simulink library "Lib_Piccolo"  (R2018b)
settings: Solver=VariableStepAuto  StartTime=0.0  StopTime=10.0  RelTol=1e-3
values from neighbouring files (symbols this model uses):
  AccelErrInt2Brakes = 0.15    [SimulationControlConfig16P.m]    (also in SimulationControlConfig16P_LEGACY.m; SimulationControlConfigTAILLESS.m = 0.2; SimulationControlConfigUTAIL.m = 0.2)
  AileronMax = 25    [SimulationControlConfig16P.m]    (also in SimulationControlConfig16P_LEGACY.m; SimulationControlConfigTAILLESS.m; SimulationControlConfigUTAIL.m)
  AileronPower = 0.00268    [SimulationControlConfig16P.m]    (also in SimulationControlConfig16P_LEGACY.m; SimulationControlConfigTAILLESS.m; SimulationControlConfigUTAIL.m)
  AileronSurfaceMax = 45    [SimulationControlConfig16P.m]    (also in SimulationControlConfig16P_LEGACY.m)
  AileronTrim = 0    [SimulationControlConfig16P.m]    (also in SimulationControlConfig16P_LEGACY.m; SimulationControlConfigTAILLESS.m; SimulationControlConfigUTAIL.m)
  Alt = 1000 + TerrainHeight    [SimulationStateConfig.m]
  AltCruise_m = testPlans(testIndx).terrainElevation * 0.3048 + 200    [SimulationControlConfig16P.m]    (also in SimulationControlConfigTAILLESS.m = 1083; SimulationControlConfigUTAIL.m = testPlans(testIndx).terrainElevation * 0.3048 + 152)
  AltitudeRate2PitchCmdIntegratorInit = 0.1    [SimulationControlPre.m]
  AltMax = 10000    [SimulationControlConfig16P.m]    (also in SimulationControlConfig16P_LEGACY.m; SimulationControlConfigTAILLESS.m; SimulationControlConfigUTAIL.m)
  AltMaxAccel = 1.25    [SimulationControlConfig16P.m]    (also in SimulationControlConfig16P_LEGACY.m = 0.9; SimulationControlConfigTAILLESS.m = 1.7; SimulationControlConfigUTAIL.m = 2)
  AltMin = 0    [SimulationControlConfig16P.m]    (also in SimulationControlConfig16P_LEGACY.m; SimulationControlConfigTAILLESS.m; SimulationControlConfigUTAIL.m)
  AltRateCmd2Pitch = 0.50    (= 0.5)    [SimulationControlConfig16P.m]    (also in SimulationControlConfig16P_LEGACY.m = 0.6; SimulationControlConfigTAILLESS.m = 0.2; SimulationControlConfigUTAIL.m = 0.3)
  AltRateError2Pitch = 0.40    (= 0.4)    [SimulationControlConfig16P.m]    (also in SimulationControlConfig16P_LEGACY.m; SimulationControlConfigTAILLESS.m = 0.55; SimulationControlConfigUTAIL.m = 0.55)
  AltRateErrorInt2Pitch = 0.50    (= 0.5)    [SimulationControlConfig16P.m]    (also in SimulationControlConfig16P_LEGACY.m = 0.45; SimulationControlConfigTAILLESS.m; SimulationControlConfigUTAIL.m = 0.75)
  AltRateLpfCutOff = 3    [SimulationControlConfig16P.m]    (also in SimulationControlConfig16P_LEGACY.m; SimulationControlConfigTAILLESS.m = 2; SimulationControlConfigUTAIL.m = 2)
  AutoNosegear2Rudder = 26    [SimulationControlConfig16P.m]    (also in SimulationControlConfig16P_LEGACY.m; SimulationControlConfigTAILLESS.m = 25.2; SimulationControlConfigUTAIL.m = 14)
  b = 5.54    [SimulationControlConfig16P.m]    (also in SimulationControlConfig16P_LEGACY.m; SimulationControlConfigTAILLESS.m = 2.37; SimulationControlConfigUTAIL.m = 2.37)
  Bank2AileronIntegratorInit = 0    [SimulationControlPre.m]
  BankMax_User = BankMax_User/180*pi    (= 0.523598775598)    [SimulationControlConfig16P.m]    (also in SimulationControlConfig16P_LEGACY.m; SimulationControlConfigTAILLESS.m = 0.610865238198; SimulationControlConfigUTAIL.m = 0.628318530718)
  baseLegFlaps = 20    [SimulationControlConfig16P.m]    (also in SimulationControlConfig16P_LEGACY.m = 0; SimulationControlConfigTAILLESS.m = 15; SimulationControlConfigUTAIL.m = 10)
  C = GeneticOpt.C    [SimulationCostFunction.m]
  c = Sw/b    (= 0.841696750903)    [SimulationControlConfig16P.m]    (also in SimulationControlConfig16P_LEGACY.m; SimulationControlConfigTAILLESS.m = 0.354008438819; SimulationControlConfigUTAIL.m = 0.354008438819)
  cell2WheelFactorMG = 5.98    [SimulationSensorConfig16P_LEGACY.m]
  cell2WheelFactorNG = 1    [SimulationSensorConfig16P_LEGACY.m]
  cellSatMaxMG = 15000    [SimulationSensorConfig16P.m]    (also in SimulationSensorConfig16P_LEGACY.m; SimulationSensorConfigTAILLESS7P.m; SimulationSensorConfigUTAIL7P.m)
  cellSatMaxNG = 1000    [SimulationSensorConfig16P.m]    (also in SimulationSensorConfig16P_LEGACY.m; SimulationSensorConfigTAILLESS7P.m; SimulationSensorConfigUTAIL7P.m)
  cellSatMinMG = -15000    [SimulationSensorConfig16P.m]    (also in SimulationSensorConfig16P_LEGACY.m; SimulationSensorConfigTAILLESS7P.m; SimulationSensorConfigUTAIL7P.m)
  cellSatMinNG = -1000    [SimulationSensorConfig16P.m]    (also in SimulationSensorConfig16P_LEGACY.m; SimulationSensorConfigTAILLESS7P.m; SimulationSensorConfigUTAIL7P.m)
  CL_Limit = CL_Max    (= 0.54)    [SimulationControlConfig16P.m]    (also in SimulationControlConfig16P_LEGACY.m; SimulationControlConfigTAILLESS.m; SimulationControlConfigUTAIL.m = 0.53)
  CL_Max = 0.54    [SimulationControlConfig16P.m]    (also in SimulationControlConfig16P_LEGACY.m; SimulationControlConfigTAILLESS.m; SimulationControlConfigUTAIL.m = 0.53)
  CL_Max_Nom = 0.465    [SimulationControlConfig16P.m]    (also in SimulationControlConfig16P_LEGACY.m; SimulationControlConfigTAILLESS.m = 0.39; SimulationControlConfigUTAIL.m)
  CL_Min = 0    [SimulationControlConfig16P.m]    (also in SimulationControlConfig16P_LEGACY.m; SimulationControlConfigTAILLESS.m; SimulationControlConfigUTAIL.m)
  ClimbMaxFraction = 0.35    [SimulationControlConfig16P.m]    (also in SimulationControlConfig16P_LEGACY.m = 0.24; SimulationControlConfigTAILLESS.m = 0.19; SimulationControlConfigUTAIL.m = 0.21)
  ClimboutMaxBank = 7.0    (= 7)    [SimulationControlConfig16P.m]    (also in SimulationControlConfig16P_LEGACY.m; SimulationControlConfigTAILLESS.m = 5; SimulationControlConfigUTAIL.m)
  ClimboutTimer = 7.0    (= 7)    [SimulationControlConfig16P.m]    (also in SimulationControlConfig16P_LEGACY.m; SimulationControlConfigTAILLESS.m; SimulationControlConfigUTAIL.m)
  dCl_per_dFlap = 0.005581818    [SimulationControlConfig16P.m]    (also in SimulationControlConfig16P_LEGACY.m = 0; SimulationControlConfigTAILLESS.m = 0; SimulationControlConfigUTAIL.m = 0)
  DecelerationCmd = 3.1    [SimulationControlConfig16P.m]    (also in SimulationControlConfig16P_LEGACY.m; SimulationControlConfigTAILLESS.m = 0.1; SimulationControlConfigUTAIL.m = 0.1)
  DeRotateLogicEndTimer = abs((NoseDownLimit_Deg-1)/DeRotateRamp_Dps)    [SimulationControlConfig16P.m]    (also in SimulationControlConfig16P_LEGACY.m; SimulationControlConfigTAILLESS.m; SimulationControlConfigUTAIL.m)
  DeRotateLogicHoldNoseUpTimer = 0.1    [SimulationControlConfig16P.m]    (also in SimulationControlConfig16P_LEGACY.m; SimulationControlConfigTAILLESS.m; SimulationControlConfigUTAIL.m)
  DeRotateLogicTimerTimeout = 2    [SimulationControlConfig16P.m]    (also in SimulationControlConfig16P_LEGACY.m; SimulationControlConfigTAILLESS.m; SimulationControlConfigUTAIL.m)
  DeRotateLowerCmdSaturation = 0    [SimulationControlConfig16P.m]    (also in SimulationControlConfig16P_LEGACY.m; SimulationControlConfigTAILLESS.m; SimulationControlConfigUTAIL.m)
  DeRotateRamp_Dps = 3    [SimulationControlConfig16P.m]    (also in SimulationControlConfig16P_LEGACY.m; SimulationControlConfigTAILLESS.m = 8; SimulationControlConfigUTAIL.m = 8)
  DeRotateUpperCmdSaturation = 7    [SimulationControlConfig16P.m]    (also in SimulationControlConfig16P_LEGACY.m; SimulationControlConfigTAILLESS.m; SimulationControlConfigUTAIL.m)
  DescentMaxFraction = 0.22    [SimulationControlConfig16P.m]    (also in SimulationControlConfig16P_LEGACY.m = 0.2; SimulationControlConfigTAILLESS.m = 0.17; SimulationControlConfigUTAIL.m = 0.17)
  DesktopSimTerrainOffset_m = 0.406    [SimulationAircraftConfig.m]
  downwindFlaps = 0    [SimulationControlConfig16P.m]    (also in SimulationControlConfig16P_LEGACY.m; SimulationControlConfigTAILLESS.m; SimulationControlConfigUTAIL.m)
  DP_init = 0.5*1.225*V_init^2    [SimulationControlConfig16P.m]    (also in SimulationControlConfig16P_LEGACY.m; SimulationControlConfigTAILLESS.m; SimulationControlConfigUTAIL.m)
  dscNoiseMG = 1    [SimulationSensorConfig16P_LEGACY.m]
  dscNoiseNG = 0.25    [SimulationSensorConfig16P_LEGACY.m]
  DSCnumBits = 24    [SimulationSensorConfig16P.m]    (also in SimulationSensorConfig16P_LEGACY.m; SimulationSensorConfigTAILLESS7P.m; SimulationSensorConfigUTAIL7P.m)
  DSCRangeMaxMG = 15000    [SimulationSensorConfig16P.m]    (also in SimulationSensorConfig16P_LEGACY.m; SimulationSensorConfigTAILLESS7P.m; SimulationSensorConfigUTAIL7P.m)
  DSCRangeMaxNG = 1000    [SimulationSensorConfig16P.m]    (also in SimulationSensorConfig16P_LEGACY.m; SimulationSensorConfigTAILLESS7P.m; SimulationSensorConfigUTAIL7P.m)
  DSCRangeMinMG = -15000    [SimulationSensorConfig16P.m]    (also in SimulationSensorConfig16P_LEGACY.m; SimulationSensorConfigTAILLESS7P.m; SimulationSensorConfigUTAIL7P.m)
  DSCRangeMinNG = -1000    [SimulationSensorConfig16P.m]    (also in SimulationSensorConfig16P_LEGACY.m; SimulationSensorConfigTAILLESS7P.m; SimulationSensorConfigUTAIL7P.m)
  dt = DLLSim.dt    [SimulationTimeStep.m]    (also in SimulationTrim.m = 0.02)
  EarlyTouchdownThreshold = 3.0    (= 3)    [SimulationControlConfig16P.m]    (also in SimulationControlConfig16P_LEGACY.m; SimulationControlConfigTAILLESS.m = 2.2; SimulationControlConfigUTAIL.m = 2.5)
  ElevatorDeflectionRate = 15    [SimulationControlConfig16P.m]    (also in SimulationControlConfig16P_LEGACY.m = 12; SimulationControlConfigTAILLESS.m = 10; SimulationControlConfigUTAIL.m = 12)
  ElevatorMax = 25    [SimulationControlConfig16P.m]    (also in SimulationControlConfig16P_LEGACY.m; SimulationControlConfigTAILLESS.m; SimulationControlConfigUTAIL.m)
  ElevatorPower = -0.002209    [SimulationControlConfig16P.m]    (also in SimulationControlConfig16P_LEGACY.m; SimulationControlConfigTAILLESS.m = -0.002956; SimulationControlConfigUTAIL.m = -0.00205983)
  ElevatorTrim = -3.5    [SimulationControlConfig16P.m]    (also in SimulationControlConfig16P_LEGACY.m; SimulationControlConfigTAILLESS.m = -6; SimulationControlConfigUTAIL.m = -8)
  elevonBias = 0    [SimulationControlConfig16P.m]    (also in SimulationControlConfig16P_LEGACY.m; SimulationControlConfigTAILLESS.m; SimulationControlConfigUTAIL.m)
  Enable_TAS_Protection = 0    [SimulationControlConfig16P.m]    (also in SimulationControlConfig16P_LEGACY.m; SimulationControlConfigTAILLESS.m; SimulationControlConfigUTAIL.m)
  EnableCrossTrackAbort = 1    [SimulationControlConfig16P.m]    (also in SimulationControlConfigTAILLESS.m; SimulationControlConfigUTAIL.m)
  EnergyBandwidth = 0.02    [SimulationControlConfig16P.m]    (also in SimulationControlConfig16P_LEGACY.m; SimulationControlConfigTAILLESS.m = 0.06; SimulationControlConfigUTAIL.m = 0.06)
  EngineLhFuelCut = 0    [SimulationAircraftConfig.m]
  EngineRhFuelCut = 0    [SimulationAircraftConfig.m]
  FastThrottleRate = 0.075    [SimulationControlConfig16P.m]    (also in SimulationControlConfig16P_LEGACY.m = 0.05; SimulationControlConfigTAILLESS.m = 0.1; SimulationControlConfigUTAIL.m = 0.1)
  FilterWarmUpTime = 2    [SimulationSensorConfig16P.m]    (also in SimulationSensorConfig16P_LEGACY.m; SimulationSensorConfigTAILLESS7P.m; SimulationSensorConfigUTAIL7P.m)
  finalApproachFlaps = 20    [SimulationControlConfig16P.m]    (also in SimulationControlConfig16P_LEGACY.m = 0; SimulationControlConfigTAILLESS.m = 22; SimulationControlConfigUTAIL.m = 10)
  FinalDescentSlope_Deg = testPlans(testIndx).descentSlope    [SimulationControlConfig16P.m]    (also in SimulationControlConfig16P_LEGACY.m; SimulationControlConfigTAILLESS.m; SimulationControlConfigUTAIL.m)
  flapMax = 0    [SimulationControlConfig16P.m]    (also in SimulationControlConfig16P_LEGACY.m; SimulationControlConfigTAILLESS.m; SimulationControlConfigUTAIL.m)
  flapRate = 7.5    [SimulationControlConfig16P.m]    (also in SimulationControlConfig16P_LEGACY.m; SimulationControlConfigTAILLESS.m = 6.6; SimulationControlConfigUTAIL.m)
  FlareHeight = 5    [SimulationControlConfig16P.m]    (also in SimulationControlConfig16P_LEGACY.m = 4.8; SimulationControlConfigTAILLESS.m = 2.5; SimulationControlConfigUTAIL.m = 2)
  FlareVerticalRate_mps = -0.4    [SimulationControlConfig16P.m]    (also in SimulationControlConfig16P_LEGACY.m = -0.5; SimulationControlConfigTAILLESS.m = -0.15; SimulationControlConfigUTAIL.m = -0.15)
  Fp_Aileron = 0.55*2*pi*RollRateLpfCutoff*dt    [SimulationControlConfig16P.m]    (also in SimulationControlConfig16P_LEGACY.m; SimulationControlConfigTAILLESS.m; SimulationControlConfigUTAIL.m)
  Fp_Alt = 0.55*AltBandwidth    (= 0.099)    [SimulationControlConfig16P.m]    (also in SimulationControlConfig16P_LEGACY.m; SimulationControlConfigTAILLESS.m = 0.587477826221; SimulationControlConfigUTAIL.m = 0.69115038379)
  Fp_AltRate = 0.55*2*pi*AltRateLpfCutOff*dt    [SimulationControlConfig16P.m]    (also in SimulationControlConfig16P_LEGACY.m; SimulationControlConfigTAILLESS.m; SimulationControlConfigUTAIL.m)
  Fp_Elevator = 0.55*2*pi*PitchRateLpfCutoff*dt    [SimulationControlConfig16P.m]    (also in SimulationControlConfig16P_LEGACY.m; SimulationControlConfigTAILLESS.m; SimulationControlConfigUTAIL.m)
  Fp_Energy = 0.55*2*pi*EnergyBandwidth    (= 0.069115038379)    [SimulationControlConfig16P.m]    (also in SimulationControlConfig16P_LEGACY.m; SimulationControlConfigTAILLESS.m = 0.207345115137; SimulationControlConfigUTAIL.m = 0.207345115137)
  Fp_Energy2 = 0.55*2*pi*EnergyBandwidth*dt    [SimulationControlConfig16P.m]    (also in SimulationControlConfig16P_LEGACY.m; SimulationControlConfigTAILLESS.m; SimulationControlConfigUTAIL.m)
  Fp_Pitch = 0.55*2*pi*PitchBandwidth    (= 2.76460153516)    [SimulationControlConfig16P.m]    (also in SimulationControlConfig16P_LEGACY.m = 3.11017672705; SimulationControlConfigTAILLESS.m = 3.80132711084; SimulationControlConfigUTAIL.m = 2.41902634326)
  Fp_Pitch_2 = 0.55*2*pi*PitchBandwidth*dt    [SimulationControlConfig16P.m]    (also in SimulationControlConfig16P_LEGACY.m; SimulationControlConfigTAILLESS.m; SimulationControlConfigUTAIL.m)
  Fp_Roll = RollBandwidth^2    (= 1)    [SimulationControlConfig16P.m]    (also in SimulationControlConfig16P_LEGACY.m = 1.44; SimulationControlConfigTAILLESS.m; SimulationControlConfigUTAIL.m)
  Fp_Rudder = 0.55*2*pi*YawRateLpfCutoff*dt    [SimulationControlConfig16P.m]    (also in SimulationControlConfig16P_LEGACY.m; SimulationControlConfigTAILLESS.m; SimulationControlConfigUTAIL.m)
  Fp_TAS = 0.55*2*pi*TASBandwidth    (= 0.103672557568)    [SimulationControlConfig16P.m]    (also in SimulationControlConfig16P_LEGACY.m; SimulationControlConfigTAILLESS.m = 0.172787595947; SimulationControlConfigUTAIL.m = 0.172787595947)
  Fp_TAS_Filter = 2*pi*TasLpfCutoff*dt    [SimulationControlConfig16P.m]    (also in SimulationControlConfig16P_LEGACY.m; SimulationControlConfigTAILLESS.m; SimulationControlConfigUTAIL.m)
  Fp_Turn = 0.55*2*pi*TurnErrLPFcutoff    (= 0.0345575191895)    [SimulationControlConfig16P.m]    (also in SimulationControlConfig16P_LEGACY.m; SimulationControlConfigTAILLESS.m = 0.172787595947; SimulationControlConfigUTAIL.m = 0.172787595947)
  Fp_TurnDerr = 0.55*2*pi*TurnDerivativeLPFcutoff    (= 0.0345575191895)    [SimulationControlConfig16P.m]    (also in SimulationControlConfig16P_LEGACY.m; SimulationControlConfigTAILLESS.m = 0.172787595947; SimulationControlConfigUTAIL.m = 0.172787595947)
  FTV = 3    [SimulationAircraftConfig.m]
  ftvStaticPositionError = 1/1.18    (= 0.847457627119)    [SimulationSensorConfig16P.m]    (also in SimulationSensorConfig16P_LEGACY.m; SimulationSensorConfigTAILLESS7P.m = 1; SimulationSensorConfigUTAIL7P.m = 1)
  g = 9.81    [SimulationStateConfig.m]
  GustSpd_Kts = testPlans(testIndx).gustSpd    [SimulationStateConfig.m]
  GustTriggerVal = testPlans(testIndx).gustTriggerVal    [SimulationStateConfig.m]
  HeadingErr2TurnRate = 0.5    [SimulationControlConfig16P.m]    (also in SimulationControlConfig16P_LEGACY.m; SimulationControlConfigTAILLESS.m; SimulationControlConfigUTAIL.m)
  HeadingErrDer2TurnRate = 0.3    [SimulationControlConfig16P.m]    (also in SimulationControlConfig16P_LEGACY.m; SimulationControlConfigTAILLESS.m; SimulationControlConfigUTAIL.m)
  IASbounce = IASstall*0.8    [SimulationControlPre.m]
  IAScruiseCMD = sqrt(2*m*9.81/(1.225*Sw*CL_cruise))    [SimulationControlConfig16P.m]    (also in SimulationControlConfig16P_LEGACY.m; SimulationControlConfigTAILLESS.m; SimulationControlConfigUTAIL.m)
  IASfinalCMD = 1.12 * IASmin    [SimulationControlConfig16P.m]    (also in SimulationControlConfig16P_LEGACY.m = 1.10 * IASmin; SimulationControlConfigTAILLESS.m = 1.10 * IASmin; SimulationControlConfigUTAIL.m = 1.15 * IASmin)
  IASflareCMD = IASstall    [SimulationControlConfig16P.m]    (also in SimulationControlConfig16P_LEGACY.m; SimulationControlConfigTAILLESS.m; SimulationControlConfigUTAIL.m)
  IASmax = 64    [SimulationControlConfig16P.m]    (also in SimulationControlConfig16P_LEGACY.m = 46; SimulationControlConfigTAILLESS.m = 38.58; SimulationControlConfigUTAIL.m = 35)
  IASmin = sqrt(2*m*9.81/(1.225*Sw*0.9*CL_Max_Nom))    [SimulationControlConfig16P.m]    (also in SimulationControlConfig16P_LEGACY.m; SimulationControlConfigTAILLESS.m; SimulationControlConfigUTAIL.m)
  IASshortCMD = IASstall    [SimulationControlConfig16P.m]    (also in SimulationControlConfig16P_LEGACY.m; SimulationControlConfigTAILLESS.m; SimulationControlConfigUTAIL.m)
  IASstall = sqrt(2*m*9.81/(1.225*Sw*CL_Max))    [SimulationControlConfig16P.m]    (also in SimulationControlConfig16P_LEGACY.m; SimulationControlConfigTAILLESS.m; SimulationControlConfigUTAIL.m)
  inFlight = 1    [SimulationControlConfig16P.m]    (also in SimulationControlConfigTAILLESS.m; SimulationControlConfigUTAIL.m)
  JetCatOffset = 5    [SimulationControlConfig16P.m]    (also in SimulationControlConfig16P_LEGACY.m)
  LaunchRollingElevator = -1.5    [SimulationControlConfig16P.m]    (also in SimulationControlConfig16P_LEGACY.m; SimulationControlConfigTAILLESS.m = 1; SimulationControlConfigUTAIL.m = 1)
  ldg_NosegearMax = 10    [SimulationControlConfig16P.m]    (also in SimulationControlConfig16P_LEGACY.m; SimulationControlConfigTAILLESS.m; SimulationControlConfigUTAIL.m)
  ldg_TrackVyErrInt2Nosegear = 0.1250    (= 0.125)    [SimulationControlConfig16P.m]    (also in SimulationControlConfig16P_LEGACY.m; SimulationControlConfigTAILLESS.m = 0.00714285714286; SimulationControlConfigUTAIL.m = 0.00714285714286)
  ldg_TrackVyErrPro2Nosegear = 0.35    [SimulationControlConfig16P.m]    (also in SimulationControlConfig16P_LEGACY.m; SimulationControlConfigTAILLESS.m = 0.0546666666667; SimulationControlConfigUTAIL.m = 0.0546666666667)
  ldg_TrackY2Vy = 0.07    [SimulationControlConfig16P.m]    (also in SimulationControlConfig16P_LEGACY.m; SimulationControlConfigTAILLESS.m = 0.17; SimulationControlConfigUTAIL.m = 0.17)
  ldg_Vy2NosegearScalingPower = 1.075    [SimulationControlConfig16P.m]    (also in SimulationControlConfig16P_LEGACY.m; SimulationControlConfigTAILLESS.m = 0.6; SimulationControlConfigUTAIL.m = 0.5)
  ldg_Y2VyScalingPower = 0.175    [SimulationControlConfig16P.m]    (also in SimulationControlConfig16P_LEGACY.m; SimulationControlConfigTAILLESS.m = 0; SimulationControlConfigUTAIL.m = 0)
  ldg_YawRate2Nosegear = 0.175    [SimulationControlConfig16P.m]    (also in SimulationControlConfig16P_LEGACY.m; SimulationControlConfigTAILLESS.m = 0.065; SimulationControlConfigUTAIL.m = 0.065)
  LiftSlope = 0.064285    [SimulationControlConfig16P.m]    (also in SimulationControlConfig16P_LEGACY.m; SimulationControlConfigTAILLESS.m = 0.058631; SimulationControlConfigUTAIL.m)
  LPFaileronInit = 0    [SimulationControlPre.m]
  LPFclestInit = 0    [SimulationControlPre.m]
  LPFenergyFFInit = 0    [SimulationControlPre.m]
  LPFtasInit = V_init + 2    [SimulationControlPre.m]
  LPFthrottleInit = ThrottleTrim    [SimulationControlPre.m]
  LPFturnErrInit = 0    [SimulationControlPre.m]
  ... (+115 more)
undefined symbols (not defined in the file or in its folder): abortFlag, alphaHPF, apmDelay, BRWNOUT, CRAWOR, CRAWUR, DiscIntNeverNeededParam, DLLSim, DLLSimStep, ECOMOR, ECOMUR, Fp_Tas, GustTrigger_HeightAgl_m, IPSTAT, LCINTEG, Ldg_Persist_Time, LOWER_FLAGS, MSG_ENABLE, NoiseStd, OLDVAL, OVERRIDE_ENABLE, OVERRIDE_VALUE, REBOOT, reversionEnable, revIASMax, revIASMin, revPitchMax, revPitchMin, revPitchRateMax, revRollMax, revRollRateMax, SAMPLE, SCALON, SensorModel, sigbuilder_block, Sim_Vx, Sim_Vy, Sim_Vz, Sim_Xpos, Sim_Ypos, Sim_Zpos, SYSOR, SYSUR, TARE, TEMPOR, TEMPUR, testIndx, testPlan, testPlans, Trim_piccoloInCmd, Trim_REFSI_FD_IN_nmodeCgShifterCmd_Ft, Trim_REFSI_FD_IN_nmodeFlapLhIBCmd_Deg, Trim_REFSI_FD_IN_nmodeFlapLhOBCmd_Deg, Trim_REFSI_FD_IN_nmodeFlapRhIBCmd_Deg, Trim_REFSI_FD_IN_nmodeFlapRhOBCmd_Deg, Trim_REFSI_FD_IN_nmodeSlatLhCmd_Deg, Trim_REFSI_FD_IN_nmodeSlatRhCmd_Deg, Trim_REFSI_FD_IN_nmodeSplrLhInbdCmd_Deg, Trim_REFSI_FD_IN_nmodeSplrLhOutbdCmd_Deg ... (+5)
libraries: simulink x866, aerolibconvert2 x60, $bdroot x52, aerolibatmos2 x5, dspswit3 x5, simulink_extras x4, dsparch4 x2, Lib_Piccolo_Alt x2, eeGeneralControl x1, dspindex x1
(part 43 of 44)

== system Lib_Piccolo/Ground Detection Systems/WoW Wrapper/Variant Subsystem/Load Cell WoW Model 20/WOW Module/Subsystem/Health Check/DSC STAT Decode ==
  MGR STAT Word : Inport
  MGL STAT Word : Inport  Port=2
  NG STAT Word : Inport  Port=3
  Bus Creator : BusCreator  Inputs=IPSTAT,TEMPUR,TEMPOR,ECOMUR,ECOMOR,CRAWUR,CRAWOR,SYSUR,SYSOR,LCINTEG,SCALON,OLDVAL  OutDataTypeStr=Bus: STAT_SIGNAL_BUS  NonVirtualBus=on
  Bus Creator1 : BusCreator  Inputs=IPSTAT,TEMPUR,TEMPOR,ECOMUR,ECOMOR,CRAWUR,CRAWOR,SYSUR,SYSOR,LCINTEG,SCALON,OLDVAL  OutDataTypeStr=Bus: STAT_SIGNAL_BUS  NonVirtualBus=on
  Bus Creator2 : BusCreator  Inputs=IPSTAT,TEMPUR,TEMPOR,ECOMUR,ECOMOR,CRAWUR,CRAWOR,SYSUR,SYSOR,LCINTEG,SCALON,OLDVAL  OutDataTypeStr=Bus: STAT_SIGNAL_BUS  NonVirtualBus=on
  Extract STAT MGL : $bdroot/Ground Detection Systems/WoW Wrapper/Variant Subsystem/Load Cell WoW Model 20/WOW Module/Subsystem/Health Check/DSC STAT Decode/Extract STAT MGR  SystemSampleTime=-1
  Extract STAT MGR : Subsystem
  Extract STAT NG : $bdroot/Ground Detection Systems/WoW Wrapper/Variant Subsystem/Load Cell WoW Model 20/WOW Module/Subsystem/Health Check/DSC STAT Decode/Extract STAT MGR  SystemSampleTime=-1
  MGR_STAT : Outport  OutDataTypeStr=Bus: STAT_SIGNAL_BUS
  MGL_STAT : Outport  Port=2  OutDataTypeStr=Bus: STAT_SIGNAL_BUS
  NG_STAT : Outport  Port=3  OutDataTypeStr=Bus: STAT_SIGNAL_BUS
  wires:
  MGR STAT Word/1 -> Extract STAT MGR/1(STAT Word)
  MGL STAT Word/1 -> Extract STAT MGL/1
  NG STAT Word/1 -> Extract STAT NG/1
  Extract STAT MGR/1(IPSTAT) -> Bus Creator/1  "IPSTAT"
  Extract STAT MGR/2(TEMPUR) -> Bus Creator/2  "TEMPUR"
  Extract STAT MGR/3(TEMPOR) -> Bus Creator/3  "TEMPOR"
  Extract STAT MGR/4(ECOMUR) -> Bus Creator/4  "ECOMUR"
  Extract STAT MGR/5(ECOMOR) -> Bus Creator/5  "ECOMOR"
  Extract STAT MGR/6(CRAWUR) -> Bus Creator/6  "CRAWUR"
  Extract STAT MGR/7(CRAWOR) -> Bus Creator/7  "CRAWOR"
  Extract STAT MGR/8(SYSUR) -> Bus Creator/8  "SYSUR"
  Extract STAT MGR/9(SYSOR) -> Bus Creator/9  "SYSOR"
  Extract STAT MGR/10(LCINTEG) -> Bus Creator/10  "LCINTEG"
  Extract STAT MGR/11(SCALON) -> Bus Creator/11  "SCALON"
  Extract STAT MGR/12(OLDVAL) -> Bus Creator/12  "OLDVAL"
  Bus Creator/1 -> MGR_STAT/1
  Extract STAT MGL/1 -> Bus Creator1/1  "IPSTAT"
  Extract STAT MGL/2 -> Bus Creator1/2  "TEMPUR"
  Extract STAT MGL/3 -> Bus Creator1/3  "TEMPOR"
  Extract STAT MGL/4 -> Bus Creator1/4  "ECOMUR"
  Extract STAT MGL/5 -> Bus Creator1/5  "ECOMOR"
  Extract STAT MGL/6 -> Bus Creator1/6  "CRAWUR"
  Extract STAT MGL/7 -> Bus Creator1/7  "CRAWOR"
  Extract STAT MGL/8 -> Bus Creator1/8  "SYSUR"
  Extract STAT MGL/9 -> Bus Creator1/9  "SYSOR"
  Extract STAT MGL/10 -> Bus Creator1/10  "LCINTEG"
  Extract STAT MGL/11 -> Bus Creator1/11  "SCALON"
  Extract STAT MGL/12 -> Bus Creator1/12  "OLDVAL"
  Bus Creator1/1 -> MGL_STAT/1
  Extract STAT NG/1 -> Bus Creator2/1  "IPSTAT"
  Extract STAT NG/2 -> Bus Creator2/2  "TEMPUR"
  Extract STAT NG/3 -> Bus Creator2/3  "TEMPOR"
  Extract STAT NG/4 -> Bus Creator2/4  "ECOMUR"
  Extract STAT NG/5 -> Bus Creator2/5  "ECOMOR"
  Extract STAT NG/6 -> Bus Creator2/6  "CRAWUR"
  Extract STAT NG/7 -> Bus Creator2/7  "CRAWOR"
  Extract STAT NG/8 -> Bus Creator2/8  "SYSUR"
  Extract STAT NG/9 -> Bus Creator2/9  "SYSOR"
  Extract STAT NG/10 -> Bus Creator2/10  "LCINTEG"
  Extract STAT NG/11 -> Bus Creator2/11  "SCALON"
  Extract STAT NG/12 -> Bus Creator2/12  "OLDVAL"
  Bus Creator2/1 -> NG_STAT/1

== system Lib_Piccolo/Ground Detection Systems/WoW Wrapper/Variant Subsystem/Load Cell WoW Model 20/WOW Module/Subsystem/Health Check/MGR DSC Fail Logic ==
  PIC_AP_MODE : Inport
  WOW_N : Inport  Port=2
  LOAD_TIMEOUT : Inport  Port=3
  FLAG_RESET : Inport  Port=4
  FLAG_TIMEOUT : Inport  Port=5
  Bus Creator : BusCreator  Inputs=8  OutDataTypeStr=Bus: HEALTH_SIGNAL_BUS  NonVirtualBus=on
  Constant : Constant  Value=0  OutDataTypeStr=boolean
  Latch : Subsystem
  Latch Activation on Mode : $bdroot/Ground Detection Systems/WoW Wrapper/Variant Subsystem/Load Cell WoW Model 20/WOW Module/Flag Latch/Latch Activation on Mode  SystemSampleTime=-1
  MG Data Validation : Subsystem
  OR3 : Logic  Operator=OR  Inputs=5  IconShape=distinctive  AllPortsSameDT=off  OutDataTypeStr=boolean
  DSC_FAIL : Outport
  MGR_HEALTH : Outport  Port=2
  wires:
  WOW_N/1 -> MG Data Validation/2(WOW_N)
  OR3/1 -> Latch/1(D)
  FLAG_RESET/1 -> Bus Creator/6, OR3/5  "FLAG_ERROR"
  MG Data Validation/1(INVALID) -> Bus Creator/1, OR3/1  "INVALID"
  Bus Creator/1 -> MGR_HEALTH/1
  LOAD_TIMEOUT/1 -> Bus Creator/4, OR3/3  "LOAD_TIMEOUT"
  MG Data Validation/2(IN_FLIGHT_BIAS) -> Bus Creator/2  "IN_FLIGHT_BIAS"
  Latch Activation on Mode/1 -> Latch/2(Enable/!Rst)
  PIC_AP_MODE/1 -> Latch Activation on Mode/1, MG Data Validation/1(AP Mode)
  Latch/1(Q_Latched) -> Bus Creator/8, DSC_FAIL/1  "FAIL"
  FLAG_TIMEOUT/1 -> Bus Creator/5, OR3/4  "FLAG_TIMEOUT"
  MG Data Validation/3(FINAL_BIAS) -> OR3/2, Bus Creator/3  "FINAL_BIAS"
  Constant/1 -> Bus Creator/7  "ACTIVE"

== system Lib_Piccolo/Ground Detection Systems/WoW Wrapper/Variant Subsystem/Load Cell WoW Model 20/WOW Module/Subsystem/Health Check/NG DSC Fail Logic ==
  PIC_AP_MODE : Inport
  WOW_N : Inport  Port=2
  LOAD_TIMEOUT : Inport  Port=3
  FLAG_RESET : Inport  Port=4
  FLAG_TIMEOUT : Inport  Port=5
  Bus Creator : BusCreator  Inputs=8  OutDataTypeStr=Bus: HEALTH_SIGNAL_BUS  NonVirtualBus=on
  Constant : Constant  Value=0  OutDataTypeStr=boolean
  Latch : Subsystem
  Latch Activation on Mode : $bdroot/Ground Detection Systems/WoW Wrapper/Variant Subsystem/Load Cell WoW Model 20/WOW Module/Flag Latch/Latch Activation on Mode  SystemSampleTime=-1
  NG Data Validation : Subsystem
  OR3 : Logic  Operator=OR  Inputs=5  IconShape=distinctive  AllPortsSameDT=off  OutDataTypeStr=boolean
  DSC_FAIL : Outport
  MGR_HEALTH : Outport  Port=2
  wires:
  WOW_N/1 -> NG Data Validation/2(WOW_N)
  OR3/1 -> Latch/1(D)
  FLAG_RESET/1 -> Bus Creator/6, OR3/5  "FLAG_ERROR"
  NG Data Validation/1(INVALID) -> Bus Creator/1, OR3/1  "INVALID"
  Bus Creator/1 -> MGR_HEALTH/1
  LOAD_TIMEOUT/1 -> Bus Creator/4, OR3/3  "LOAD_TIMEOUT"
  NG Data Validation/2(IN_FLIGHT_BIAS) -> Bus Creator/2  "IN_FLIGHT_BIAS"
  Latch Activation on Mode/1 -> Latch/2(Enable/!Rst)
  PIC_AP_MODE/1 -> Latch Activation on Mode/1, NG Data Validation/1(AP Mode)
  Latch/1(Q_Latched) -> Bus Creator/8, DSC_FAIL/1  "FAIL"
  FLAG_TIMEOUT/1 -> Bus Creator/5, OR3/4  "FLAG_TIMEOUT"
  NG Data Validation/3(FINAL_BIAS) -> OR3/2, Bus Creator/3  "FINAL_BIAS"
  Constant/1 -> Bus Creator/7  "ACTIVE"

== system Lib_Piccolo/Ground Detection Systems/WoW Wrapper/Variant Subsystem/Load Cell WoW Model 20/WOW Module/Subsystem/Comms Timeout Logic/FLAG Timeout Counter/Custom Counter ==
  note: Custom counter with initial condition exposed as an input.
  Inc : Inport  OutDataTypeStr=boolean
  Rst : Inport  Port=2  OutDataTypeStr=boolean
  Init : Inport  Port=3  OutDataTypeStr=uint8
  Data Type Conversion : DataTypeConversion  OutDataTypeStr=uint8
  Memory : Memory  InitialCondition=SensorModel.WOW.Cell.FLAG_TIMEOUT_COUNTS
  Sum : Sum  Inputs=|++
  Switch : Switch  Criteria=u2 > Threshold  Threshold=0.5
  Cnt : Outport  OutDataTypeStr=uint8
  wires:
  Data Type Conversion/1 -> Sum/1
  Sum/1 -> Switch/3
  Rst/1 -> Switch/2
  Switch/1 -> Cnt/1, Memory/1
  Init/1 -> Switch/1
  Memory/1 -> Sum/2
  Inc/1 -> Data Type Conversion/1

== system Lib_Piccolo/Ground Detection Systems/WoW Wrapper/Variant Subsystem/Load Cell WoW Model 20/WOW Module/Subsystem/Comms Timeout Logic/LOAD Timeout Counter/Custom Counter ==
  note: Custom counter with initial condition exposed as an input.
  Inc : Inport  OutDataTypeStr=boolean
  Rst : Inport  Port=2  OutDataTypeStr=boolean
  Init : Inport  Port=3  OutDataTypeStr=uint8
  Data Type Conversion : DataTypeConversion  OutDataTypeStr=uint8
  Memory : Memory  InitialCondition=SensorModel.WOW.Cell.LOAD_TIMEOUT_COUNTS
  Sum : Sum  Inputs=|++
  Switch : Switch  Criteria=u2 > Threshold  Threshold=0.5
  Cnt : Outport  OutDataTypeStr=uint8
  wires:
  Inc/1 -> Data Type Conversion/1
  Memory/1 -> Sum/2
  Init/1 -> Switch/1
  Switch/1 -> Memory/1, Cnt/1
  Rst/1 -> Switch/2
  Sum/1 -> Switch/3
  Data Type Conversion/1 -> Sum/1

== system Lib_Piccolo/Ground Detection Systems/WoW Wrapper/Variant Subsystem/Load Cell WoW Model 20/WOW Module/Subsystem/Comms Timeout Logic/LOAD Timeout Counter/Limit Count ==
  note: If timeout condition has already been met, and trigger input is still active, dont increment the counter further.
      |
      | This prevents the counter from free-running during a sustained trigger condition, so we can use an 8-bit datatype without worrying about overflow.
  Timeout : Inport
  Trigger : Inport  Port=2
  AND : Logic  IconShape=distinctive  AllPortsSameDT=off  OutDataTypeStr=boolean
  Constant : Constant  Value=0  OutDataTypeStr=boolean
  Switch : Switch  Criteria=u2 > Threshold  Threshold=0.5
  Unit Delay : UnitDelay  SampleTime=-1
  Inc : Outport
  wires:
  Unit Delay/1 -> AND/1
  Trigger/1 -> Switch/3, AND/2
  Constant/1 -> Switch/1
  AND/1 -> Switch/2
  Timeout/1 -> Unit Delay/1
  Switch/1 -> Inc/1

== system Lib_Piccolo/Ground Detection Systems/WoW Wrapper/Variant Subsystem/Load Cell WoW Model 20/WOW Module/Subsystem/Health Check/DSC FLAG Decode/Extract Flags MGR ==
  note: Check if any critical flags set, excluding reserved bits.
  note: Bit - Function
      | 0 - Reserved
      | 1 - Reserved
      | 2 - Temp Under-Range
      | 3 - Temp Over-Range
      | 4 - Strain Gauge Input Under-Range
      | 5 - Strain Gauge Input Over-Range
      | 6 - Cell Under-Range
      | 7 - Cell Over-Range
      | 8 - System Under-Range
      | 9 - System Over-Range
      | 10 - Reserved
      | 11 - Load Cell Integrity Error
      | 12 - Watchdog Reset
      | 13 - Reserved
      | 14 - Brown-Out Reset
      | 15 - Reboot Warning (Normal Power-Up)
  Flag Word : Inport  OutDataTypeStr=uint16
  Data Type Conversion{,1..15} (16 alike) : DataTypeConversion  OutDataTypeStr=boolean
  Extract Bits : simulink/Logic and Bit Operations/Extract Bits  bitsToExtract=Range of bits  numBits=8  bitIdxRange=[0 0]  outScalingMode=Treat bit field as an integer
      settings: SourceProductName=Simulink
  Extract Bits1 : simulink/Logic and Bit Operations/Extract Bits  bitsToExtract=Range of bits  numBits=8  bitIdxRange=[1 1]  outScalingMode=Treat bit field as an integer
      settings: SourceProductName=Simulink
  Extract Bits10 : simulink/Logic and Bit Operations/Extract Bits  bitsToExtract=Range of bits  numBits=8  bitIdxRange=[10 10]  outScalingMode=Treat bit field as an integer
      settings: SourceProductName=Simulink
  Extract Bits11 : simulink/Logic and Bit Operations/Extract Bits  bitsToExtract=Range of bits  numBits=8  bitIdxRange=[11 11]  outScalingMode=Treat bit field as an integer
      settings: SourceProductName=Simulink
  Extract Bits12 : simulink/Logic and Bit Operations/Extract Bits  bitsToExtract=Range of bits  numBits=8  bitIdxRange=[12 12]  outScalingMode=Treat bit field as an integer
      settings: SourceProductName=Simulink
  Extract Bits13 : simulink/Logic and Bit Operations/Extract Bits  bitsToExtract=Range of bits  numBits=8  bitIdxRange=[13 13]  outScalingMode=Treat bit field as an integer
      settings: SourceProductName=Simulink
  Extract Bits14 : simulink/Logic and Bit Operations/Extract Bits  bitsToExtract=Range of bits  numBits=8  bitIdxRange=[14 14]  outScalingMode=Treat bit field as an integer
      settings: SourceProductName=Simulink
  Extract Bits15 : simulink/Logic and Bit Operations/Extract Bits  bitsToExtract=Range of bits  numBits=8  bitIdxRange=[15 15]  outScalingMode=Treat bit field as an integer
      settings: SourceProductName=Simulink
  Extract Bits16 : simulink/Logic and Bit Operations/Extract Bits  bitsToExtract=Range of bits  numBits=8  bitIdxRange=[2 9]  outScalingMode=Treat bit field as an integer
      settings: SourceProductName=Simulink
  Extract Bits17 : simulink/Logic and Bit Operations/Extract Bits  bitsToExtract=Range of bits  numBits=8  bitIdxRange=[11 12]  outScalingMode=Treat bit field as an integer
      settings: SourceProductName=Simulink
  Extract Bits18 : simulink/Logic and Bit Operations/Extract Bits  bitsToExtract=Range of bits  numBits=8  bitIdxRange=[14 15]  outScalingMode=Treat bit field as an integer
      settings: SourceProductName=Simulink
  Extract Bits2 : simulink/Logic and Bit Operations/Extract Bits  bitsToExtract=Range of bits  numBits=8  bitIdxRange=[2 2]  outScalingMode=Treat bit field as an integer
      settings: SourceProductName=Simulink
  Extract Bits3 : simulink/Logic and Bit Operations/Extract Bits  bitsToExtract=Range of bits  numBits=8  bitIdxRange=[3 3]  outScalingMode=Treat bit field as an integer
      settings: SourceProductName=Simulink
  Extract Bits4 : simulink/Logic and Bit Operations/Extract Bits  bitsToExtract=Range of bits  numBits=8  bitIdxRange=[4 4]  outScalingMode=Treat bit field as an integer
      settings: SourceProductName=Simulink
  Extract Bits5 : simulink/Logic and Bit Operations/Extract Bits  bitsToExtract=Range of bits  numBits=8  bitIdxRange=[5 5]  outScalingMode=Treat bit field as an integer
      settings: SourceProductName=Simulink
  Extract Bits6 : simulink/Logic and Bit Operations/Extract Bits  bitsToExtract=Range of bits  numBits=8  bitIdxRange=[6 6]  outScalingMode=Treat bit field as an integer
      settings: SourceProductName=Simulink
  Extract Bits7 : simulink/Logic and Bit Operations/Extract Bits  bitsToExtract=Range of bits  numBits=8  bitIdxRange=[7 7]  outScalingMode=Treat bit field as an integer
      settings: SourceProductName=Simulink
  Extract Bits8 : simulink/Logic and Bit Operations/Extract Bits  bitsToExtract=Range of bits  numBits=8  bitIdxRange=[8 8]  outScalingMode=Treat bit field as an integer
      settings: SourceProductName=Simulink
  Extract Bits9 : simulink/Logic and Bit Operations/Extract Bits  bitsToExtract=Range of bits  numBits=8  bitIdxRange=[9 9]  outScalingMode=Treat bit field as an integer
      settings: SourceProductName=Simulink
  OR : Logic  Operator=OR  Inputs=3  IconShape=distinctive  AllPortsSameDT=off  OutDataTypeStr=boolean
  Terminator{,1..3} (4 alike) : Terminator
  TEMPUR : Outport  OutDataTypeStr=boolean
  TEMPOR : Outport  Port=2  OutDataTypeStr=boolean
  ECOMUR : Outport  Port=3  OutDataTypeStr=boolean
  ECOMOR : Outport  Port=4  OutDataTypeStr=boolean
  CRAWUR : Outport  Port=5  OutDataTypeStr=boolean
  CRAWOR : Outport  Port=6  OutDataTypeStr=boolean
  SYSUR : Outport  Port=7  OutDataTypeStr=boolean
  SYSOR : Outport  Port=8  OutDataTypeStr=boolean
  LCINTEG : Outport  Port=9  OutDataTypeStr=boolean
  WDRST : Outport  Port=10  OutDataTypeStr=boolean
  BRWNOUT : Outport  Port=11  OutDataTypeStr=boolean
  REBOOT : Outport  Port=12  OutDataTypeStr=boolean
  LOWER_FLAGS : Outport  Port=13  OutDataTypeStr=boolean
  wires:
  Extract Bits14/1 -> Data Type Conversion14/1
  Extract Bits6/1 -> Data Type Conversion6/1
  Extract Bits12/1 -> Data Type Conversion12/1
  Extract Bits4/1 -> Data Type Conversion4/1
  Extract Bits5/1 -> Data Type Conversion5/1
  Extract Bits2/1 -> Data Type Conversion2/1
  Extract Bits/1 -> Data Type Conversion/1
  Extract Bits15/1 -> Data Type Conversion15/1
  Extract Bits13/1 -> Data Type Conversion13/1
  Extract Bits7/1 -> Data Type Conversion7/1
  Extract Bits8/1 -> Data Type Conversion8/1
  Extract Bits9/1 -> Data Type Conversion9/1
  Extract Bits1/1 -> Data Type Conversion1/1
  Extract Bits11/1 -> Data Type Conversion11/1
  Extract Bits10/1 -> Data Type Conversion10/1
  Extract Bits3/1 -> Data Type Conversion3/1
  Flag Word/1 -> Extract Bits15/1, Extract Bits14/1, Extract Bits13/1, Extract Bits12/1, Extract Bits11/1, Extract Bits10/1, Extract Bits9/1, Extract Bits8/1, Extract Bits7/1, Extract Bits6/1, Extract Bits5/1, Extract Bits4/1, Extract Bits3/1, Extract Bits2/1, Extract Bits1/1, Extract Bits16/1, Extract Bits17/1, Extract Bits18/1, Extract Bits/1
  Extract Bits17/1 -> OR/2
  Extract Bits16/1 -> OR/1
  Extract Bits18/1 -> OR/3
  OR/1 -> LOWER_FLAGS/1
  Data Type Conversion/1 -> Terminator/1
  Data Type Conversion1/1 -> Terminator1/1
  Data Type Conversion2/1 -> TEMPUR/1
  Data Type Conversion3/1 -> TEMPOR/1
  Data Type Conversion4/1 -> ECOMUR/1
  Data Type Conversion5/1 -> ECOMOR/1
  Data Type Conversion6/1 -> CRAWUR/1
  Data Type Conversion7/1 -> CRAWOR/1
  Data Type Conversion8/1 -> SYSUR/1
  Data Type Conversion9/1 -> SYSOR/1
  Data Type Conversion10/1 -> Terminator2/1
  Data Type Conversion11/1 -> LCINTEG/1
  Data Type Conversion12/1 -> WDRST/1
  Data Type Conversion13/1 -> Terminator3/1
  Data Type Conversion14/1 -> BRWNOUT/1
  Data Type Conversion15/1 -> REBOOT/1

== system Lib_Piccolo/Ground Detection Systems/WoW Wrapper/Variant Subsystem/Load Cell WoW Model 20/WOW Module/Subsystem/Health Check/DSC FLAG Decode/Persistence Counter ==
  Trigger/!Rst : Inport  OutDataTypeStr=boolean
  Compare To Constant : simulink/Logic and Bit Operations/Compare To Constant  relop=>=  const=SensorModel.WOW.Cell.FLAG_COUNTS  OutDataTypeStr=boolean
  Counter : dspswit3/Counter  Direction=Up  CountEvent=Non-zero sample  CounterSize=8 bits  MaxCount=10  InitialCount=0  Output=Count  HitValue=32  ResetInput=on  SamplesPerFrame=1  Ts=1  CntDtype=uint8  HitDtype=Logical
  Limit Count : $bdroot/Ground Detection Systems/WoW Wrapper/Variant Subsystem/Load Cell WoW Model 20/WOW Module/Subsystem/Comms Timeout Logic/LOAD Timeout Counter/Limit Count  SystemSampleTime=-1
  NOT : Logic  Operator=NOT  IconShape=distinctive  AllPortsSameDT=off  OutDataTypeStr=boolean
  TIMEOUT : Outport
  wires:
  Counter/1 -> Compare To Constant/1
  Compare To Constant/1 -> TIMEOUT/1, Limit Count/1
  NOT/1 -> Counter/2
  Trigger/!Rst/1 -> NOT/1, Limit Count/2
  Limit Count/1 -> Counter/1

== system Lib_Piccolo/Ground Detection Systems/WoW Wrapper/Variant Subsystem/Load Cell WoW Model 20/WOW Module/Subsystem/Health Check/DSC STAT Decode/Extract STAT MGR ==
  note: Bit - Function
      | 0 - Reserved
      | 1 - Digital Input Status
      | 2 - Temp Under-Range
      | 3 - Temp Over-Range
      | 4 - Strain Gauge Input Under-Range
      | 5 - Strain Gauge Input Over-Range
      | 6 - Cell Under-Range
      | 7 - Cell Over-Range
      | 8 - System Under-Range
      | 9 - System Over-Range
      | 10 - Reserved
      | 11 - Load Cell Integrity Error
      | 12 - Shunt Calibration Resistor ON
      | 13 - Shunt Output Value Previously Read
      | 14 - Reserved
      | 15 - Reserved
  STAT Word : Inport  OutDataTypeStr=uint16
  Data Type Conversion{,1..15} (16 alike) : DataTypeConversion  OutDataTypeStr=boolean
  Extract Bits : simulink/Logic and Bit Operations/Extract Bits  bitsToExtract=Range of bits  numBits=8  bitIdxRange=[0 0]  outScalingMode=Treat bit field as an integer
      settings: SourceProductName=Simulink
  Extract Bits1 : simulink/Logic and Bit Operations/Extract Bits  bitsToExtract=Range of bits  numBits=8  bitIdxRange=[1 1]  outScalingMode=Treat bit field as an integer
      settings: SourceProductName=Simulink
  Extract Bits10 : simulink/Logic and Bit Operations/Extract Bits  bitsToExtract=Range of bits  numBits=8  bitIdxRange=[10 10]  outScalingMode=Treat bit field as an integer
      settings: SourceProductName=Simulink
  Extract Bits11 : simulink/Logic and Bit Operations/Extract Bits  bitsToExtract=Range of bits  numBits=8  bitIdxRange=[11 11]  outScalingMode=Treat bit field as an integer
      settings: SourceProductName=Simulink
  Extract Bits12 : simulink/Logic and Bit Operations/Extract Bits  bitsToExtract=Range of bits  numBits=8  bitIdxRange=[12 12]  outScalingMode=Treat bit field as an integer
      settings: SourceProductName=Simulink
  Extract Bits13 : simulink/Logic and Bit Operations/Extract Bits  bitsToExtract=Range of bits  numBits=8  bitIdxRange=[13 13]  outScalingMode=Treat bit field as an integer
      settings: SourceProductName=Simulink
  Extract Bits14 : simulink/Logic and Bit Operations/Extract Bits  bitsToExtract=Range of bits  numBits=8  bitIdxRange=[14 14]  outScalingMode=Treat bit field as an integer
      settings: SourceProductName=Simulink
  Extract Bits15 : simulink/Logic and Bit Operations/Extract Bits  bitsToExtract=Range of bits  numBits=8  bitIdxRange=[15 15]  outScalingMode=Treat bit field as an integer
      settings: SourceProductName=Simulink
  Extract Bits2 : simulink/Logic and Bit Operations/Extract Bits  bitsToExtract=Range of bits  numBits=8  bitIdxRange=[2 2]  outScalingMode=Treat bit field as an integer
      settings: SourceProductName=Simulink
  Extract Bits3 : simulink/Logic and Bit Operations/Extract Bits  bitsToExtract=Range of bits  numBits=8  bitIdxRange=[3 3]  outScalingMode=Treat bit field as an integer
      settings: SourceProductName=Simulink
  Extract Bits4 : simulink/Logic and Bit Operations/Extract Bits  bitsToExtract=Range of bits  numBits=8  bitIdxRange=[4 4]  outScalingMode=Treat bit field as an integer
      settings: SourceProductName=Simulink
  Extract Bits5 : simulink/Logic and Bit Operations/Extract Bits  bitsToExtract=Range of bits  numBits=8  bitIdxRange=[5 5]  outScalingMode=Treat bit field as an integer
      settings: SourceProductName=Simulink
  Extract Bits6 : simulink/Logic and Bit Operations/Extract Bits  bitsToExtract=Range of bits  numBits=8  bitIdxRange=[6 6]  outScalingMode=Treat bit field as an integer
      settings: SourceProductName=Simulink
  Extract Bits7 : simulink/Logic and Bit Operations/Extract Bits  bitsToExtract=Range of bits  numBits=8  bitIdxRange=[7 7]  outScalingMode=Treat bit field as an integer
      settings: SourceProductName=Simulink
  Extract Bits8 : simulink/Logic and Bit Operations/Extract Bits  bitsToExtract=Range of bits  numBits=8  bitIdxRange=[8 8]  outScalingMode=Treat bit field as an integer
      settings: SourceProductName=Simulink
  Extract Bits9 : simulink/Logic and Bit Operations/Extract Bits  bitsToExtract=Range of bits  numBits=8  bitIdxRange=[9 9]  outScalingMode=Treat bit field as an integer
      settings: SourceProductName=Simulink
  Terminator{,1..3} (4 alike) : Terminator
  IPSTAT : Outport  OutDataTypeStr=boolean
  TEMPUR : Outport  Port=2  OutDataTypeStr=boolean
  TEMPOR : Outport  Port=3  OutDataTypeStr=boolean
  ECOMUR : Outport  Port=4  OutDataTypeStr=boolean
  ECOMOR : Outport  Port=5  OutDataTypeStr=boolean
  CRAWUR : Outport  Port=6  OutDataTypeStr=boolean
  CRAWOR : Outport  Port=7  OutDataTypeStr=boolean
  SYSUR : Outport  Port=8  OutDataTypeStr=boolean
  SYSOR : Outport  Port=9  OutDataTypeStr=boolean
  LCINTEG : Outport  Port=10  OutDataTypeStr=boolean
  SCALON : Outport  Port=11  OutDataTypeStr=boolean
  OLDVAL : Outport  Port=12  OutDataTypeStr=boolean
  wires:
  Extract Bits14/1 -> Data Type Conversion14/1
  Extract Bits6/1 -> Data Type Conversion6/1
  Extract Bits12/1 -> Data Type Conversion12/1
  Extract Bits4/1 -> Data Type Conversion4/1
  Extract Bits5/1 -> Data Type Conversion5/1
  Extract Bits2/1 -> Data Type Conversion2/1
  Extract Bits/1 -> Data Type Conversion/1
  Extract Bits15/1 -> Data Type Conversion15/1
  Extract Bits13/1 -> Data Type Conversion13/1
  Extract Bits7/1 -> Data Type Conversion7/1
  Extract Bits8/1 -> Data Type Conversion8/1
  Extract Bits9/1 -> Data Type Conversion9/1
  Extract Bits1/1 -> Data Type Conversion1/1
  Extract Bits11/1 -> Data Type Conversion11/1
  Extract Bits10/1 -> Data Type Conversion10/1
  Extract Bits3/1 -> Data Type Conversion3/1
  STAT Word/1 -> Extract Bits15/1, Extract Bits14/1, Extract Bits13/1, Extract Bits12/1, Extract Bits11/1, Extract Bits10/1, Extract Bits9/1, Extract Bits8/1, Extract Bits7/1, Extract Bits6/1, Extract Bits5/1, Extract Bits4/1, Extract Bits3/1, Extract Bits2/1, Extract Bits1/1, Extract Bits/1
  Data Type Conversion/1 -> Terminator/1
  Data Type Conversion1/1 -> IPSTAT/1
  Data Type Conversion2/1 -> TEMPUR/1
  Data Type Conversion3/1 -> TEMPOR/1
  Data Type Conversion4/1 -> ECOMUR/1
  Data Type Conversion5/1 -> ECOMOR/1
  Data Type Conversion6/1 -> CRAWUR/1
  Data Type Conversion7/1 -> CRAWOR/1
  Data Type Conversion8/1 -> SYSUR/1
  Data Type Conversion9/1 -> SYSOR/1
  Data Type Conversion10/1 -> Terminator2/1
  Data Type Conversion11/1 -> LCINTEG/1
  Data Type Conversion12/1 -> SCALON/1
  Data Type Conversion13/1 -> OLDVAL/1
  Data Type Conversion14/1 -> Terminator1/1
  Data Type Conversion15/1 -> Terminator3/1

== system Lib_Piccolo/Ground Detection Systems/WoW Wrapper/Variant Subsystem/Load Cell WoW Model 20/WOW Module/Subsystem/Health Check/MGR DSC Fail Logic/Latch ==
  D : Inport
  Enable/!Rst : Inport  Port=2
  AND : Logic  IconShape=distinctive  AllPortsSameDT=off  OutDataTypeStr=boolean
  Constant : Constant  OutDataTypeStr=boolean
  OR : Logic  Operator=OR  IconShape=distinctive  AllPortsSameDT=off  OutDataTypeStr=boolean
  Switch : Switch  Criteria=u2 > Threshold  Threshold=0.5
  Unit Delay : UnitDelay  SampleTime=-1
  Q_Latched : Outport
  wires:
  Constant/1 -> Switch/1
  Enable/!Rst/1 -> AND/2
  AND/1 -> Switch/2
  OR/1 -> AND/1
  D/1 -> OR/1, Switch/3
  Switch/1 -> Unit Delay/1, Q_Latched/1
  Unit Delay/1 -> OR/2

== system Lib_Piccolo/Ground Detection Systems/WoW Wrapper/Variant Subsystem/Load Cell WoW Model 20/WOW Module/Subsystem/Health Check/MGR DSC Fail Logic/MG Data Validation ==
  AP Mode : Inport
  WOW_N : Inport  Port=2
  AND : Logic  IconShape=distinctive  AllPortsSameDT=off  OutDataTypeStr=boolean
  AND1 : Logic  IconShape=distinctive  AllPortsSameDT=off  OutDataTypeStr=boolean
  Abs : Abs
  Compare To Constant : simulink/Logic and Bit Operations/Compare To Constant  relop=>  const=SensorModel.WOW.Cell.satMaxMGWheel  OutDataTypeStr=boolean
  Compare To Constant1 : simulink/Logic and Bit Operations/Compare To Constant  relop=<  const=SensorModel.WOW.Cell.satMinMGWheel  OutDataTypeStr=boolean
  Compare To Constant2 : simulink/Logic and Bit Operations/Compare To Constant  relop=>  const=SensorModel.WOW.Cell.loadThresholdLower_N  OutDataTypeStr=boolean
  Greater Than Climbout : simulink/Logic and Bit Operations/Compare To Constant  relop=>  const=3  OutDataTypeStr=boolean
  Is on Final : simulink/Logic and Bit Operations/Compare To Constant  relop===  const=8  OutDataTypeStr=boolean
  Less Than Final Mode : simulink/Logic and Bit Operations/Compare To Constant  relop=<  const=8  OutDataTypeStr=boolean
  OR : Logic  Operator=OR  IconShape=distinctive  AllPortsSameDT=off  OutDataTypeStr=boolean
  OR1 : Logic  IconShape=distinctive  AllPortsSameDT=off  OutDataTypeStr=boolean
  Persistence Counter : Subsystem
  Persistence Counter1 : $bdroot/Ground Detection Systems/WoW Wrapper/Variant Subsystem/Load Cell WoW Model 20/WOW Module/Subsystem/Health Check/MGR DSC Fail Logic/MG Data Validation/Persistence Counter  SystemSampleTime=-1
  Persistence Counter2 : $bdroot/Ground Detection Systems/WoW Wrapper/Variant Subsystem/Load Cell WoW Model 20/WOW Module/Subsystem/Health Check/MGR DSC Fail Logic/MG Data Validation/Persistence Counter  SystemSampleTime=-1
  INVALID : Outport
  IN_FLIGHT_BIAS : Outport  Port=2
  FINAL_BIAS : Outport  Port=3
  wires:
  WOW_N/1 -> Compare To Constant/1, Abs/1, Compare To Constant1/1
  Compare To Constant/1 -> OR/1
  Compare To Constant1/1 -> OR/2
  OR/1 -> Persistence Counter/1(Trigger/!Rst)
  Persistence Counter/1(TIMEOUT) -> INVALID/1
  Persistence Counter1/1 -> IN_FLIGHT_BIAS/1
  AP Mode/1 -> Is on Final/1, Greater Than Climbout/1, Less Than Final Mode/1
  Compare To Constant2/1 -> AND1/2, AND/2
  AND/1 -> Persistence Counter1/1
  OR1/1 -> AND/1
  Less Than Final Mode/1 -> OR1/2
  Greater Than Climbout/1 -> OR1/1
  Persistence Counter2/1 -> FINAL_BIAS/1
  AND1/1 -> Persistence Counter2/1
  Is on Final/1 -> AND1/1
  Abs/1 -> Compare To Constant2/1

== system Lib_Piccolo/Ground Detection Systems/WoW Wrapper/Variant Subsystem/Load Cell WoW Model 20/WOW Module/Subsystem/Health Check/NG DSC Fail Logic/Latch ==
  D : Inport
  Enable/!Rst : Inport  Port=2
  AND : Logic  IconShape=distinctive  AllPortsSameDT=off  OutDataTypeStr=boolean
  Constant : Constant  OutDataTypeStr=boolean
  OR : Logic  Operator=OR  IconShape=distinctive  AllPortsSameDT=off  OutDataTypeStr=boolean
  Switch : Switch  Criteria=u2 > Threshold  Threshold=0.5
  Unit Delay : UnitDelay  SampleTime=-1
  Q_Latched : Outport
  wires:
  Constant/1 -> Switch/1
  Enable/!Rst/1 -> AND/2
  AND/1 -> Switch/2
  OR/1 -> AND/1
  D/1 -> OR/1, Switch/3
  Switch/1 -> Unit Delay/1, Q_Latched/1
  Unit Delay/1 -> OR/2
